simulink model "dcmotorACFC"  (R2022b)
settings: Solver=ode23s  StartTime=0.0  StopTime=10  RelTol=1e-3
settings Model: Creator=Admin_EEE  LastModifiedBy=Admin_EEE

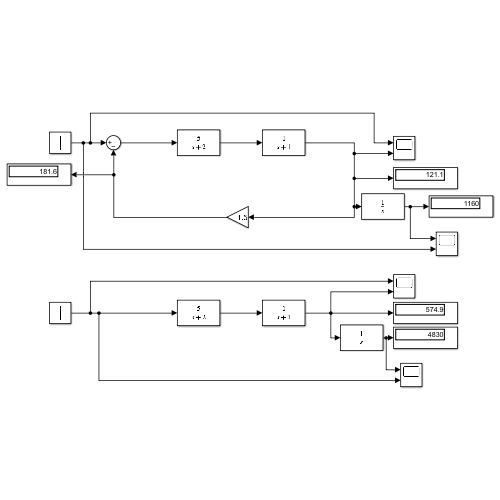
[thumbnail: Simulink's stored preview of the top-level diagram]
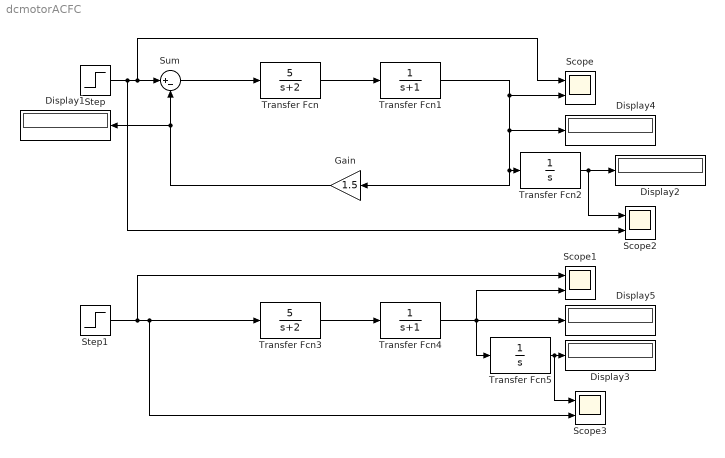
== system dcmotorACFC ==
  Display{1..5} (5 alike) : Display
  Gain : Gain  Gain=1.5
  Scope{,1..3} (4 alike) : Scope  NumInputPorts=2
  Step : Step  Time=0.1  After=230  SampleTime=0
  Step1 : Step  Time=0.1  After=230  SampleTime=0
  Sum : Sum  Inputs=|+-
  Transfer Fcn : TransferFcn  Numerator=[5]  Denominator=[1 2]
  Transfer Fcn1 : TransferFcn  Denominator=[1 1]
  Transfer Fcn2 : TransferFcn  Denominator=[1 0]
  Transfer Fcn3 : TransferFcn  Numerator=[5]  Denominator=[1 2]
  Transfer Fcn4 : TransferFcn  Denominator=[1 1]
  Transfer Fcn5 : TransferFcn  Denominator=[1 0]
  wires:
  Step/1 -> Scope2/2, Scope/1, Sum/1
  Sum/1 -> Transfer Fcn/1
  Transfer Fcn/1 -> Transfer Fcn1/1
  Transfer Fcn1/1 -> Display4/1, Gain/1, Transfer Fcn2/1, Scope/2
  Gain/1 -> Display1/1, Sum/2
  Transfer Fcn2/1 -> Scope2/1, Display2/1
  Transfer Fcn4/1 -> Transfer Fcn5/1, Display5/1, Scope1/2
  Transfer Fcn3/1 -> Transfer Fcn4/1
  Transfer Fcn5/1 -> Scope3/1, Display3/1
  Step1/1 -> Scope3/2, Transfer Fcn3/1, Scope1/1
